simulink library "sm_wheel_loader_lib"  (R2025a)
settings: Solver=VariableStepAuto  StartTime=0.0  StopTime=10.0  RelTol=1e-3
undefined symbols (not defined in the file): AToTOrificeVector, BiPOrificeVector, boomHEArea, boomREArea, BToTOrificeVector, fluids, GRake, GToothL, GToothR, HMPST, HydFcnParams, logLoad, Position, PToAOrificeVector, PToBOrificeVector, RakeL, RakeR, testInput, Wheel_Loader, X, Y, Z
libraries: sm_lib x694, fl_lib x183, nesl_utility x74, SimscapeFluids_lib x62, sdl_lib x25, cvt_components_lib x25, simulink_extras x5, $bdroot x4, wheel_loader_contact_lib x4, ee_lib x2, SignalEditorBlockLib x1, batteryecm_lib x1
(part 12 of 26)

== system sm_wheel_loader_lib/Wheel Loader Vehicle/Frame Front/Lights/Cap Front ==
  Cap_Front : sm_lib/Body Elements/File Solid  ExtGeomFileName=FrameF_Cap_Front.step  UnitType=FromFile  ExtGeomFileUnits=m  StepReaderType=HEX  ExportConvexHullGeometry=off  InertiaType=Custom  BasedOnType=DensityFromFile  Density=1000  DensityUnits=kg/m^3  Mass=0.394195570353179  MassUnits=lbm  CenterOfMass=[0 18.9709186614173 25.112965984252]  CenterOfMassUnits=in  MomentsOfInertia=[0.29984658255218 0.29984658255218 0.584592682486173]  MomentsOfInertiaUnits=lbm*in^2  ProductsOfInertia=[0 0 0]  ProductsOfInertiaUnits=lbm*in^2  GraphicType=FromGeometry  MarkerShape=Sphere  MarkerSize=10  GraphicVisPropType=SimpleVisualProperties  GraphicDiffuseColor=[0.196078431 0.196078431 0.196078431]  GraphicOpacity=HMPST.Vis.Cap.opc  GraphicSpecularColor=[0.5 0.5 0.5 1.0]  GraphicAmbientColor=[0.15 0.15 0.15 1.0]  GraphicEmissiveColor=[0.0 0.0 0.0 1.0]  GraphicShininess=75  DoExposeReferenceFrame=on  SerializedFrames=<Frames/>
  Transform : sm_lib/Frames and Transforms/Rigid Transform  RotationMethod=ArbitraryAxis  FollAlignAxisA=+X  BaseAlignAxisA=+Y  FollAlignAxisB=+Y  BaseAlignAxisB=+Z  RotationStandardAxis=+Z  RotationAngle=0  RotationAngleUnits=rad  RotationArbitraryAxis=[0 0 0]  RotationSequenceAxes=FollowerAxes  RotationSequence=XYX  RotationSequenceAngles=[0 0 0]  RotationSequenceAnglesUnits=deg  RotationMatrix=[1 0 0; 0 1 0; 0 0 1]  Quaternion=[1 0 0 0]  TranslationMethod=Cartesian  TranslationCartesianOffset=[0 18.9709186614173 25.1378139370079]  TranslationCartesianOffsetUnits=in  TranslationStandardAxis=+Z  TranslationStandardOffset=0  TranslationStandardOffsetUnits=m  TranslationROffset=0  TranslationROffsetUnits=m  TranslationThetaOffset=0  TranslationThetaOffsetUnits=deg  TranslationZOffset=0  TranslationZOffsetUnits=m
  F : PMIOPort  Side=Left
  connections:
  Transform/RConn1 -- F/RConn1
  Cap_Front/RConn1 -- Transform/LConn1

== system sm_wheel_loader_lib/Wheel Loader Vehicle/Frame Front/Lights/Cap Side ==
  Cap_Side : sm_lib/Body Elements/File Solid  ExtGeomFileName=FrameF_Cap_Side.step  UnitType=FromFile  ExtGeomFileUnits=m  StepReaderType=HEX  ExportConvexHullGeometry=off  InertiaType=Custom  BasedOnType=DensityFromFile  Density=1000  DensityUnits=kg/m^3  Mass=0.326703632602991  MassUnits=lbm  CenterOfMass=[13.2699581496063 13.7324941732283 22.6905788976378]  CenterOfMassUnits=in  MomentsOfInertia=[0.25784270557939 0.189027697893249 0.286762231353936]  MomentsOfInertiaUnits=lbm*in^2  ProductsOfInertia=[0 0.0820087083851274 0]  ProductsOfInertiaUnits=lbm*in^2  GraphicType=FromGeometry  MarkerShape=Sphere  MarkerSize=10  GraphicVisPropType=SimpleVisualProperties  GraphicDiffuseColor=[0.901960784 0.901960784 0.901960784]  GraphicOpacity=HMPST.Vis.Cap.opc  GraphicSpecularColor=[0.5 0.5 0.5 1.0]  GraphicAmbientColor=[0.15 0.15 0.15 1.0]  GraphicEmissiveColor=[0.0 0.0 0.0 1.0]  GraphicShininess=75  DoExposeReferenceFrame=on  SerializedFrames=<Frames/>
  Transform : sm_lib/Frames and Transforms/Rigid Transform  RotationMethod=ArbitraryAxis  FollAlignAxisA=+X  BaseAlignAxisA=+Y  FollAlignAxisB=+Y  BaseAlignAxisB=+Z  RotationStandardAxis=+Z  RotationAngle=0  RotationAngleUnits=rad  RotationArbitraryAxis=[0 0 0]  RotationSequenceAxes=FollowerAxes  RotationSequence=XYX  RotationSequenceAngles=[0 0 0]  RotationSequenceAnglesUnits=deg  RotationMatrix=[1 0 0; 0 1 0; 0 0 1]  Quaternion=[1 0 0 0]  TranslationMethod=Cartesian  TranslationCartesianOffset=[29.4805690551181 -102.631127086614 57.6446281496063]  TranslationCartesianOffsetUnits=in  TranslationStandardAxis=+Z  TranslationStandardOffset=0  TranslationStandardOffsetUnits=m  TranslationROffset=0  TranslationROffsetUnits=m  TranslationThetaOffset=0  TranslationThetaOffsetUnits=deg  TranslationZOffset=0  TranslationZOffsetUnits=m
  G : PMIOPort  Side=Left
  connections:
  Transform/LConn1 -- G/RConn1
  Cap_Side/RConn1 -- Transform/RConn1

== system sm_wheel_loader_lib/Wheel Loader Vehicle/Frame Front/Lights/Light Left ==
  Housing : sm_lib/Body Elements/File Solid  ExtGeomFileName=LightF_Housing.step  UnitType=FromFile  ExtGeomFileUnits=m  StepReaderType=HEX  ExportConvexHullGeometry=off  InertiaType=Custom  BasedOnType=DensityFromFile  Density=1000  DensityUnits=kg/m^3  Mass=5.82907417512336  MassUnits=lbm  CenterOfMass=[-16.4284857874016 16.6341196850394 33.5621000393701]  CenterOfMassUnits=in  MomentsOfInertia=[45.900348235786 54.0150653364011 28.9269786264561]  MomentsOfInertiaUnits=lbm*in^2  ProductsOfInertia=[2.18871568666261 0.00164024251114051 -0.000652679832557995]  ProductsOfInertiaUnits=lbm*in^2  GraphicType=FromGeometry  MarkerShape=Sphere  MarkerSize=10  GraphicVisPropType=SimpleVisualProperties  GraphicDiffuseColor=[0.196078431 0.196078431 0.196078431]  GraphicOpacity=HMPST.Vis.Light.opc  GraphicSpecularColor=[0.5 0.5 0.5 1.0]  GraphicAmbientColor=[0.15 0.15 0.15 1.0]  GraphicEmissiveColor=[0.0 0.0 0.0 1.0]  GraphicShininess=75  DoExposeReferenceFrame=on  SerializedFrames=<Frames/>
  Inner_Reflector : sm_lib/Body Elements/File Solid  ExtGeomFileName=LightF_Inner_Reflector.step  UnitType=FromFile  ExtGeomFileUnits=m  StepReaderType=HEX  ExportConvexHullGeometry=off  InertiaType=Custom  BasedOnType=DensityFromFile  Density=1000  DensityUnits=kg/m^3  Mass=2.3813985010374  MassUnits=lbm  CenterOfMass=[-16.4286011417323 16.7992054724409 33.5198841732283]  CenterOfMassUnits=in  MomentsOfInertia=[16.7215889666979 21.0139771829924 9.91006504421532]  MomentsOfInertiaUnits=lbm*in^2  ProductsOfInertia=[0.553287970726677 -0.00263122236162124 0.000146938391623004]  ProductsOfInertiaUnits=lbm*in^2  GraphicType=FromGeometry  MarkerShape=Sphere  MarkerSize=10  GraphicVisPropType=SimpleVisualProperties  GraphicDiffuseColor=[1 1 1]  GraphicOpacity=HMPST.Vis.Light.opc  GraphicSpecularColor=[0.5 0.5 0.5 1.0]  GraphicAmbientColor=[0.15 0.15 0.15 1.0]  GraphicEmissiveColor=[0.0 0.0 0.0 1.0]  GraphicShininess=75  DoExposeReferenceFrame=on  SerializedFrames=<Frames/>
  Lens_Lower : sm_lib/Body Elements/File Solid  ExtGeomFileName=LightF_Lens_Lower.step  UnitType=FromFile  ExtGeomFileUnits=m  StepReaderType=HEX  ExportConvexHullGeometry=off  InertiaType=Custom  BasedOnType=DensityFromFile  Density=1000  DensityUnits=kg/m^3  Mass=0.955755653473624  MassUnits=lbm  CenterOfMass=[-16.4285714566929 18.8369745669291 32.0841470472441]  CenterOfMassUnits=in  MomentsOfInertia=[4.86310718087393 7.40813821570663 2.55427790198926]  MomentsOfInertiaUnits=lbm*in^2  ProductsOfInertia=[0.0290562126504745 0.000252870720467496 1.36686875928376e-05]  ProductsOfInertiaUnits=lbm*in^2  GraphicType=FromGeometry  MarkerShape=Sphere  MarkerSize=10  GraphicVisPropType=SimpleVisualProperties  GraphicDiffuseColor=[0.701960784 0.701960784 0.701960784]  GraphicOpacity=HMPST.Vis.Light.opc  GraphicSpecularColor=[0.5 0.5 0.5 1.0]  GraphicAmbientColor=[0.15 0.15 0.15 1.0]  GraphicEmissiveColor=[0.0 0.0 0.0 1.0]  GraphicShininess=75  DoExposeReferenceFrame=on  SerializedFrames=<Frames/>
  Lens_Upper : sm_lib/Body Elements/File Solid  ExtGeomFileName=LightF_Lens_Upper.step  UnitType=FromFile  ExtGeomFileUnits=m  StepReaderType=HEX  ExportConvexHullGeometry=off  InertiaType=Custom  BasedOnType=DensityFromFile  Density=1000  DensityUnits=kg/m^3  Mass=0.688422318479475  MassUnits=lbm  CenterOfMass=[-16.4285475590551 18.8615080708661 35.1565936614173]  CenterOfMassUnits=in  MomentsOfInertia=[0.831387671318652 2.25205980213972 1.42246614606763]  MomentsOfInertiaUnits=lbm*in^2  ProductsOfInertia=[0 -6.8343437964188e-06 0]  ProductsOfInertiaUnits=lbm*in^2  GraphicType=FromGeometry  MarkerShape=Sphere  MarkerSize=10  GraphicVisPropType=SimpleVisualProperties  GraphicDiffuseColor=[0.901960784 0.901960784 0.901960784]  GraphicOpacity=HMPST.Vis.Lens.opc  GraphicSpecularColor=[0.5 0.5 0.5 1.0]  GraphicAmbientColor=[0.15 0.15 0.15 1.0]  GraphicEmissiveColor=[0.0 0.0 0.0 1.0]  GraphicShininess=75  DoExposeReferenceFrame=on  SerializedFrames=<Frames/>
  Transform{,1..3} (4 alike) : sm_lib/Frames and Transforms/Rigid Transform  RotationMethod=ArbitraryAxis  FollAlignAxisA=+X  BaseAlignAxisA=+Y  FollAlignAxisB=+Y  BaseAlignAxisB=+Z  RotationStandardAxis=+Z  RotationAngle=0  RotationAngleUnits=rad  RotationArbitraryAxis=[0 0 0]  RotationSequenceAxes=FollowerAxes  RotationSequence=XYX  RotationSequenceAngles=[0 0 0]  RotationSequenceAnglesUnits=deg  RotationMatrix=[1 0 0; 0 1 0; 0 0 1]  Quaternion=[1 0 0 0]  TranslationMethod=Cartesian  TranslationCartesianOffset=[29.4805690551181 -102.631127086614 57.6446281496063]  TranslationCartesianOffsetUnits=in  TranslationStandardAxis=+Z  TranslationStandardOffset=0  TranslationStandardOffsetUnits=m  TranslationROffset=0  TranslationROffsetUnits=m  TranslationThetaOffset=0  TranslationThetaOffsetUnits=deg  TranslationZOffset=0  TranslationZOffsetUnits=m
  Transform4 : sm_lib/Frames and Transforms/Rigid Transform  RotationMethod=ArbitraryAxis  FollAlignAxisA=+X  BaseAlignAxisA=+Y  FollAlignAxisB=+Y  BaseAlignAxisB=+Z  RotationStandardAxis=+Z  RotationAngle=1.5707963267949  RotationAngleUnits=rad  RotationArbitraryAxis=[-1 0 0]  RotationSequenceAxes=FollowerAxes  RotationSequence=XYX  RotationSequenceAngles=[0 0 0]  RotationSequenceAnglesUnits=deg  RotationMatrix=[1 0 0; 0 1 0; 0 0 1]  Quaternion=[1 0 0 0]  TranslationMethod=Cartesian  TranslationCartesianOffset=[-16.4285533858268 13.4490081889764 34.3374097244095]  TranslationCartesianOffsetUnits=in  TranslationStandardAxis=+Z  TranslationStandardOffset=0  TranslationStandardOffsetUnits=m  TranslationROffset=0  TranslationROffsetUnits=m  TranslationThetaOffset=0  TranslationThetaOffsetUnits=deg  TranslationZOffset=0  TranslationZOffsetUnits=m
  F : PMIOPort  Side=Left
  connections:
  Transform3/RConn1 -- Transform4/LConn1 -- Housing/RConn1
  Lens_Lower/RConn1 -- Transform2/RConn1
  Lens_Upper/RConn1 -- Transform1/RConn1
  Inner_Reflector/RConn1 -- Transform/RConn1
  Transform4/RConn1 -- F/RConn1
  Transform3/LConn1 -- Transform2/LConn1 -- Transform1/LConn1 -- Transform/LConn1

== system sm_wheel_loader_lib/Wheel Loader Vehicle/Frame Front/Lights/Light Right ==
  Inner_Reflector : sm_lib/Body Elements/File Solid  ExtGeomFileName=LightF_Inner_Reflector.step  UnitType=FromFile  ExtGeomFileUnits=m  StepReaderType=HEX  ExportConvexHullGeometry=off  InertiaType=Custom  BasedOnType=DensityFromFile  Density=1000  DensityUnits=kg/m^3  Mass=2.3813985010374  MassUnits=lbm  CenterOfMass=[-16.4286011417323 16.7992054724409 33.5198841732283]  CenterOfMassUnits=in  MomentsOfInertia=[16.7215889666979 21.0139771829924 9.91006504421532]  MomentsOfInertiaUnits=lbm*in^2  ProductsOfInertia=[0.553287970726677 -0.00263122236162124 0.000146938391623004]  ProductsOfInertiaUnits=lbm*in^2  GraphicType=FromGeometry  MarkerShape=Sphere  MarkerSize=10  GraphicVisPropType=SimpleVisualProperties  GraphicDiffuseColor=[1 1 1]  GraphicOpacity=HMPST.Vis.Light.opc  GraphicSpecularColor=[0.5 0.5 0.5 1.0]  GraphicAmbientColor=[0.15 0.15 0.15 1.0]  GraphicEmissiveColor=[0.0 0.0 0.0 1.0]  GraphicShininess=75  DoExposeReferenceFrame=on  SerializedFrames=<Frames/>
  Lens_Lower : sm_lib/Body Elements/File Solid  ExtGeomFileName=LightF_Lens_Lower.step  UnitType=FromFile  ExtGeomFileUnits=m  StepReaderType=HEX  ExportConvexHullGeometry=off  InertiaType=Custom  BasedOnType=DensityFromFile  Density=1000  DensityUnits=kg/m^3  Mass=0.955755653473624  MassUnits=lbm  CenterOfMass=[-16.4285714566929 18.8369745669291 32.0841470472441]  CenterOfMassUnits=in  MomentsOfInertia=[4.86310718087393 7.40813821570663 2.55427790198926]  MomentsOfInertiaUnits=lbm*in^2  ProductsOfInertia=[0.0290562126504745 0.000252870720467496 1.36686875928376e-05]  ProductsOfInertiaUnits=lbm*in^2  GraphicType=FromGeometry  MarkerShape=Sphere  MarkerSize=10  GraphicVisPropType=SimpleVisualProperties  GraphicDiffuseColor=[0.701960784 0.701960784 0.701960784]  GraphicOpacity=HMPST.Vis.Light.opc  GraphicSpecularColor=[0.5 0.5 0.5 1.0]  GraphicAmbientColor=[0.15 0.15 0.15 1.0]  GraphicEmissiveColor=[0.0 0.0 0.0 1.0]  GraphicShininess=75  DoExposeReferenceFrame=on  SerializedFrames=<Frames/>
  Lens_Upper : sm_lib/Body Elements/File Solid  ExtGeomFileName=LightF_Lens_Upper.step  UnitType=FromFile  ExtGeomFileUnits=m  StepReaderType=HEX  ExportConvexHullGeometry=off  InertiaType=Custom  BasedOnType=DensityFromFile  Density=1000  DensityUnits=kg/m^3  Mass=0.688422318479475  MassUnits=lbm  CenterOfMass=[-16.4285475590551 18.8615080708661 35.1565936614173]  CenterOfMassUnits=in  MomentsOfInertia=[0.831387671318652 2.25205980213972 1.42246614606763]  MomentsOfInertiaUnits=lbm*in^2  ProductsOfInertia=[0 -6.8343437964188e-06 0]  ProductsOfInertiaUnits=lbm*in^2  GraphicType=FromGeometry  MarkerShape=Sphere  MarkerSize=10  GraphicVisPropType=SimpleVisualProperties  GraphicDiffuseColor=[0.901960784 0.901960784 0.901960784]  GraphicOpacity=HMPST.Vis.Lens.opc  GraphicSpecularColor=[0.5 0.5 0.5 1.0]  GraphicAmbientColor=[0.15 0.15 0.15 1.0]  GraphicEmissiveColor=[0.0 0.0 0.0 1.0]  GraphicShininess=75  DoExposeReferenceFrame=on  SerializedFrames=<Frames/>
  Solid : sm_lib/Body Elements/File Solid  ExtGeomFileName=LightF_Housing.step  UnitType=FromFile  ExtGeomFileUnits=m  StepReaderType=HEX  ExportConvexHullGeometry=off  InertiaType=Custom  BasedOnType=DensityFromFile  Density=1000  DensityUnits=kg/m^3  Mass=5.82907417512336  MassUnits=lbm  CenterOfMass=[-16.4284857874016 16.6341196850394 33.5621000393701]  CenterOfMassUnits=in  MomentsOfInertia=[45.900348235786 54.0150653364011 28.9269786264561]  MomentsOfInertiaUnits=lbm*in^2  ProductsOfInertia=[2.18871568666261 0.00164024251114051 -0.000652679832557995]  ProductsOfInertiaUnits=lbm*in^2  GraphicType=FromGeometry  MarkerShape=Sphere  MarkerSize=10  GraphicVisPropType=SimpleVisualProperties  GraphicDiffuseColor=[0.196078431 0.196078431 0.196078431]  GraphicOpacity=HMPST.Vis.Light.opc  GraphicSpecularColor=[0.5 0.5 0.5 1.0]  GraphicAmbientColor=[0.15 0.15 0.15 1.0]  GraphicEmissiveColor=[0.0 0.0 0.0 1.0]  GraphicShininess=75  DoExposeReferenceFrame=on  SerializedFrames=<Frames/>
  Transform{,1..3} (4 alike) : sm_lib/Frames and Transforms/Rigid Transform  RotationMethod=ArbitraryAxis  FollAlignAxisA=+X  BaseAlignAxisA=+Y  FollAlignAxisB=+Y  BaseAlignAxisB=+Z  RotationStandardAxis=+Z  RotationAngle=0  RotationAngleUnits=rad  RotationArbitraryAxis=[0 0 0]  RotationSequenceAxes=FollowerAxes  RotationSequence=XYX  RotationSequenceAngles=[0 0 0]  RotationSequenceAnglesUnits=deg  RotationMatrix=[1 0 0; 0 1 0; 0 0 1]  Quaternion=[1 0 0 0]  TranslationMethod=Cartesian  TranslationCartesianOffset=[62.3376758661417 -102.631127086614 57.6446281496063]  TranslationCartesianOffsetUnits=in  TranslationStandardAxis=+Z  TranslationStandardOffset=0  TranslationStandardOffsetUnits=m  TranslationROffset=0  TranslationROffsetUnits=m  TranslationThetaOffset=0  TranslationThetaOffsetUnits=deg  TranslationZOffset=0  TranslationZOffsetUnits=m
  Transform4 : sm_lib/Frames and Transforms/Rigid Transform  RotationMethod=ArbitraryAxis  FollAlignAxisA=+X  BaseAlignAxisA=+Y  FollAlignAxisB=+Y  BaseAlignAxisB=+Z  RotationStandardAxis=+Z  RotationAngle=1.5707963267949  RotationAngleUnits=rad  RotationArbitraryAxis=[-1 0 0]  RotationSequenceAxes=FollowerAxes  RotationSequence=XYX  RotationSequenceAngles=[0 0 0]  RotationSequenceAnglesUnits=deg  RotationMatrix=[1 0 0; 0 1 0; 0 0 1]  Quaternion=[1 0 0 0]  TranslationMethod=Cartesian  TranslationCartesianOffset=[-16.4285533858268 13.4490081889764 34.3374097244095]  TranslationCartesianOffsetUnits=in  TranslationStandardAxis=+Z  TranslationStandardOffset=0  TranslationStandardOffsetUnits=m  TranslationROffset=0  TranslationROffsetUnits=m  TranslationThetaOffset=0  TranslationThetaOffsetUnits=deg  TranslationZOffset=0  TranslationZOffsetUnits=m
  F : PMIOPort  Side=Left
  connections:
  Transform4/LConn1 -- Transform3/RConn1 -- Solid/RConn1
  Inner_Reflector/RConn1 -- Transform2/RConn1
  Lens_Upper/RConn1 -- Transform1/RConn1
  Lens_Lower/RConn1 -- Transform/RConn1
  Transform4/RConn1 -- F/RConn1
  Transform3/LConn1 -- Transform2/LConn1 -- Transform1/LConn1 -- Transform/LConn1

== system sm_wheel_loader_lib/Wheel Loader Vehicle/Frame Rear/Handles Panels/Side Handles ==
  HandleL : sm_lib/Body Elements/File Solid  ExtGeomFileName=Cab_HandleL.step  UnitType=FromFile  ExtGeomFileUnits=m  StepReaderType=HEX  ExportConvexHullGeometry=off  InertiaType=Custom  BasedOnType=DensityFromFile  Density=1000  DensityUnits=kg/m^3  Mass=6.28305972166154  MassUnits=lbm  CenterOfMass=[-17.3045312204724 -39.1271442913386 31.4849240944882]  CenterOfMassUnits=in  MomentsOfInertia=[212.912574457631 25.500464180277 191.478835295835]  MomentsOfInertiaUnits=lbm*in^2  ProductsOfInertia=[38.7009923887161 4.44232346767222e-05 -0.000140104047826585]  ProductsOfInertiaUnits=lbm*in^2  GraphicType=FromGeometry  MarkerShape=Sphere  MarkerSize=10  GraphicVisPropType=SimpleVisualProperties  GraphicDiffuseColor=[0.301960784 0.301960784 0.301960784]  GraphicOpacity=HMPST.Vis.SeatTrim.opc  GraphicSpecularColor=[0.5 0.5 0.5 1.0]  GraphicAmbientColor=[0.15 0.15 0.15 1.0]  GraphicEmissiveColor=[0.0 0.0 0.0 1.0]  GraphicShininess=75  DoExposeReferenceFrame=on  SerializedFrames=<Frames/>
  HandleR : sm_lib/Body Elements/File Solid  ExtGeomFileName=Cab_HandleR.step  UnitType=FromFile  ExtGeomFileUnits=m  StepReaderType=HEX  ExportConvexHullGeometry=off  InertiaType=Custom  BasedOnType=DensityFromFile  Density=1000  DensityUnits=kg/m^3  Mass=6.28305972166154  MassUnits=lbm  CenterOfMass=[17.3045238976378 -39.1271442913386 31.4849240944882]  CenterOfMassUnits=in  MomentsOfInertia=[212.912574457631 25.500464180277 191.478835295835]  MomentsOfInertiaUnits=lbm*in^2  ProductsOfInertia=[38.7009923887161 4.44232346767222e-05 -0.000140104047826585]  ProductsOfInertiaUnits=lbm*in^2  GraphicType=FromGeometry  MarkerShape=Sphere  MarkerSize=10  GraphicVisPropType=SimpleVisualProperties  GraphicDiffuseColor=[0.301960784 0.301960784 0.301960784]  GraphicOpacity=HMPST.Vis.SeatTrim.opc  GraphicSpecularColor=[0.5 0.5 0.5 1.0]  GraphicAmbientColor=[0.15 0.15 0.15 1.0]  GraphicEmissiveColor=[0.0 0.0 0.0 1.0]  GraphicShininess=75  DoExposeReferenceFrame=on  SerializedFrames=<Frames/>
  Transform : sm_lib/Frames and Transforms/Rigid Transform  RotationMethod=ArbitraryAxis  FollAlignAxisA=+X  BaseAlignAxisA=+Y  FollAlignAxisB=+Y  BaseAlignAxisB=+Z  RotationStandardAxis=+Z  RotationAngle=0  RotationAngleUnits=rad  RotationArbitraryAxis=[0 0 0]  RotationSequenceAxes=FollowerAxes  RotationSequence=XYX  RotationSequenceAngles=[0 0 0]  RotationSequenceAnglesUnits=deg  RotationMatrix=[1 0 0; 0 1 0; 0 0 1]  Quaternion=[1 0 0 0]  TranslationMethod=Cartesian  TranslationCartesianOffset=[-7.89410114173228 5.59542992125984 -19.0696908267717]  TranslationCartesianOffsetUnits=in  TranslationStandardAxis=+Z  TranslationStandardOffset=0  TranslationStandardOffsetUnits=m  TranslationROffset=0  TranslationROffsetUnits=m  TranslationThetaOffset=0  TranslationThetaOffsetUnits=deg  TranslationZOffset=0  TranslationZOffsetUnits=m
  Transform1 : sm_lib/Frames and Transforms/Rigid Transform  RotationMethod=ArbitraryAxis  FollAlignAxisA=+X  BaseAlignAxisA=+Y  FollAlignAxisB=+Y  BaseAlignAxisB=+Z  RotationStandardAxis=+Z  RotationAngle=0.218166156574323  RotationAngleUnits=rad  RotationArbitraryAxis=[-1 0 0]  RotationSequenceAxes=FollowerAxes  RotationSequence=XYX  RotationSequenceAngles=[0 0 0]  RotationSequenceAnglesUnits=deg  RotationMatrix=[1 0 0; 0 1 0; 0 0 1]  Quaternion=[1 0 0 0]  TranslationMethod=Cartesian  TranslationCartesianOffset=[-17.3045275590551 -39.3975186614173 30.2634644094488]  TranslationCartesianOffsetUnits=in  TranslationStandardAxis=+Z  TranslationStandardOffset=0  TranslationStandardOffsetUnits=m  TranslationROffset=0  TranslationROffsetUnits=m  TranslationThetaOffset=0  TranslationThetaOffsetUnits=deg  TranslationZOffset=0  TranslationZOffsetUnits=m
  Transform2 : sm_lib/Frames and Transforms/Rigid Transform  RotationMethod=ArbitraryAxis  FollAlignAxisA=+X  BaseAlignAxisA=+Y  FollAlignAxisB=+Y  BaseAlignAxisB=+Z  RotationStandardAxis=+Z  RotationAngle=0  RotationAngleUnits=rad  RotationArbitraryAxis=[0 0 0]  RotationSequenceAxes=FollowerAxes  RotationSequence=XYX  RotationSequenceAngles=[0 0 0]  RotationSequenceAnglesUnits=deg  RotationMatrix=[1 0 0; 0 1 0; 0 0 1]  Quaternion=[1 0 0 0]  TranslationMethod=Cartesian  TranslationCartesianOffset=[-7.89410114173228 5.59542992125984 -19.0696908267717]  TranslationCartesianOffsetUnits=in  TranslationStandardAxis=+Z  TranslationStandardOffset=0  TranslationStandardOffsetUnits=m  TranslationROffset=0  TranslationROffsetUnits=m  TranslationThetaOffset=0  TranslationThetaOffsetUnits=deg  TranslationZOffset=0  TranslationZOffsetUnits=m
  F : PMIOPort  Side=Left
  connections:
  Transform2/RConn1 -- HandleL/RConn1 -- Transform1/LConn1
  HandleR/RConn1 -- Transform/RConn1
  Transform1/RConn1 -- F/RConn1
  Transform2/LConn1 -- Transform/LConn1

== system sm_wheel_loader_lib/Wheel Loader Vehicle/Frame Rear/Handles Panels/Side Panels ==
  SeatTrimOuterL : sm_lib/Body Elements/File Solid  ExtGeomFileName=Cab_SeatTrimOuterL.step  UnitType=FromFile  ExtGeomFileUnits=m  StepReaderType=HEX  ExportConvexHullGeometry=off  InertiaType=Custom  BasedOnType=DensityFromFile  Density=1000  DensityUnits=kg/m^3  Mass=4.87052143315374  MassUnits=lbm  CenterOfMass=[-19.8295275590551 -43.9655751574803 25.4392532283465]  CenterOfMassUnits=in  MomentsOfInertia=[209.666978760431 31.2673620706489 178.412297814697]  MomentsOfInertiaUnits=lbm*in^2  ProductsOfInertia=[-6.07990400190403 0 0]  ProductsOfInertiaUnits=lbm*in^2  GraphicType=FromGeometry  MarkerShape=Sphere  MarkerSize=10  GraphicVisPropType=SimpleVisualProperties  GraphicDiffuseColor=[0.196078431 0.196078431 0.196078431]  GraphicOpacity=HMPST.Vis.SeatTrim.opc  GraphicSpecularColor=[0.5 0.5 0.5 1.0]  GraphicAmbientColor=[0.15 0.15 0.15 1.0]  GraphicEmissiveColor=[0.0 0.0 0.0 1.0]  GraphicShininess=75  DoExposeReferenceFrame=on  SerializedFrames=<Frames/>
  SeatTrimOuterR : sm_lib/Body Elements/File Solid  ExtGeomFileName=Cab_SeatTrimOuterR.step  UnitType=FromFile  ExtGeomFileUnits=m  StepReaderType=HEX  ExportConvexHullGeometry=off  InertiaType=Custom  BasedOnType=DensityFromFile  Density=1000  DensityUnits=kg/m^3  Mass=4.87052143315374  MassUnits=lbm  CenterOfMass=[19.8295275590551 -43.9655751574803 25.4392532283465]  CenterOfMassUnits=in  MomentsOfInertia=[209.666978760431 31.2673620706489 178.412297814697]  MomentsOfInertiaUnits=lbm*in^2  ProductsOfInertia=[-6.07990400190403 0 0]  ProductsOfInertiaUnits=lbm*in^2  GraphicType=FromGeometry  MarkerShape=Sphere  MarkerSize=10  GraphicVisPropType=SimpleVisualProperties  GraphicDiffuseColor=[0.196078431 0.196078431 0.196078431]  GraphicOpacity=HMPST.Vis.SeatTrim.opc  GraphicSpecularColor=[0.5 0.5 0.5 1.0]  GraphicAmbientColor=[0.15 0.15 0.15 1.0]  GraphicEmissiveColor=[0.0 0.0 0.0 1.0]  GraphicShininess=75  DoExposeReferenceFrame=on  SerializedFrames=<Frames/>
  Transform : sm_lib/Frames and Transforms/Rigid Transform  RotationMethod=ArbitraryAxis  FollAlignAxisA=+X  BaseAlignAxisA=+Y  FollAlignAxisB=+Y  BaseAlignAxisB=+Z  RotationStandardAxis=+Z  RotationAngle=0  RotationAngleUnits=rad  RotationArbitraryAxis=[0 0 0]  RotationSequenceAxes=FollowerAxes  RotationSequence=XYX  RotationSequenceAngles=[0 0 0]  RotationSequenceAnglesUnits=deg  RotationMatrix=[1 0 0; 0 1 0; 0 0 1]  Quaternion=[1 0 0 0]  TranslationMethod=Cartesian  TranslationCartesianOffset=[-7.89410114173228 5.59542992125984 -19.0696908267717]  TranslationCartesianOffsetUnits=in  TranslationStandardAxis=+Z  TranslationStandardOffset=0  TranslationStandardOffsetUnits=m  TranslationROffset=0  TranslationROffsetUnits=m  TranslationThetaOffset=0  TranslationThetaOffsetUnits=deg  TranslationZOffset=0  TranslationZOffsetUnits=m
  Transform1 : sm_lib/Frames and Transforms/Rigid Transform  RotationMethod=ArbitraryAxis  FollAlignAxisA=+X  BaseAlignAxisA=+Y  FollAlignAxisB=+Y  BaseAlignAxisB=+Z  RotationStandardAxis=+Z  RotationAngle=2.0943951023932  RotationAngleUnits=rad  RotationArbitraryAxis=[0.577350269189626 0.577350269189626 0.577350269189626]  RotationSequenceAxes=FollowerAxes  RotationSequence=XYX  RotationSequenceAngles=[0 0 0]  RotationSequenceAnglesUnits=deg  RotationMatrix=[1 0 0; 0 1 0; 0 0 1]  Quaternion=[1 0 0 0]  TranslationMethod=Cartesian  TranslationCartesianOffset=[19.7670275590551 -43.9655751574803 25.4392532283465]  TranslationCartesianOffsetUnits=in  TranslationStandardAxis=+Z  TranslationStandardOffset=0  TranslationStandardOffsetUnits=m  TranslationROffset=0  TranslationROffsetUnits=m  TranslationThetaOffset=0  TranslationThetaOffsetUnits=deg  TranslationZOffset=0  TranslationZOffsetUnits=m
  Transform2 : sm_lib/Frames and Transforms/Rigid Transform  RotationMethod=ArbitraryAxis  FollAlignAxisA=+X  BaseAlignAxisA=+Y  FollAlignAxisB=+Y  BaseAlignAxisB=+Z  RotationStandardAxis=+Z  RotationAngle=0  RotationAngleUnits=rad  RotationArbitraryAxis=[0 0 0]  RotationSequenceAxes=FollowerAxes  RotationSequence=XYX  RotationSequenceAngles=[0 0 0]  RotationSequenceAnglesUnits=deg  RotationMatrix=[1 0 0; 0 1 0; 0 0 1]  Quaternion=[1 0 0 0]  TranslationMethod=Cartesian  TranslationCartesianOffset=[-7.89410114173228 5.59542992125984 -19.0696908267717]  TranslationCartesianOffsetUnits=in  TranslationStandardAxis=+Z  TranslationStandardOffset=0  TranslationStandardOffsetUnits=m  TranslationROffset=0  TranslationROffsetUnits=m  TranslationThetaOffset=0  TranslationThetaOffsetUnits=deg  TranslationZOffset=0  TranslationZOffsetUnits=m
  F : PMIOPort  Side=Left
  connections:
  Transform2/RConn1 -- Transform1/LConn1 -- SeatTrimOuterR/RConn1
  SeatTrimOuterL/RConn1 -- Transform/RConn1
  Transform1/RConn1 -- F/RConn1
  Transform2/LConn1 -- Transform/LConn1

== system sm_wheel_loader_lib/Wheel Loader Vehicle/Linkage/Implement/Bucket ==
  Bus Element In1 : Inport  PortName=Cmd
  Bucket : Subsystem  Tag=97CFEBBA-90A8-4A4C-AFF6-5F2FCDFBD586
      mask Display: image('sm_wheel_loader_vehicle_bucket_IMAGE.png')
  Bus Creator : BusCreator  Inputs=7
  Constant{,1..6} (7 alike) : Constant  Value=0
  Simscape Bus : SimscapeBus  HierarchyStrings=Bottom
  Terminator : Terminator
  Act : PMIOPort  Side=Right
  Link : PMIOPort  Port=2  Side=Left
  Arm : PMIOPort  Port=3  Side=Left
  GImpl : PMIOPort  Port=4  Side=Right
  m : Outport
  wires:
  Constant5/1 -> Bus Creator/2  "vL"
  Constant6/1 -> Bus Creator/6  "vR"
  Constant4/1 -> Bus Creator/7  "pR"
  Bus Creator/1 -> m/1
  Constant3/1 -> Bus Creator/3  "pL"
  Constant2/1 -> Bus Creator/4  "power"
  Constant1/1 -> Bus Creator/5  "forceR"
  Constant/1 -> Bus Creator/1  "forceL"
  Bus Element In1/1 -> Terminator/1
  connections:
  Bucket/RConn1 -- Simscape Bus/LConn1
  GImpl/RConn1 -- Simscape Bus/RConn1
  Arm/RConn1 -- Bucket/LConn2
  Bucket/LConn1 -- Link/RConn1

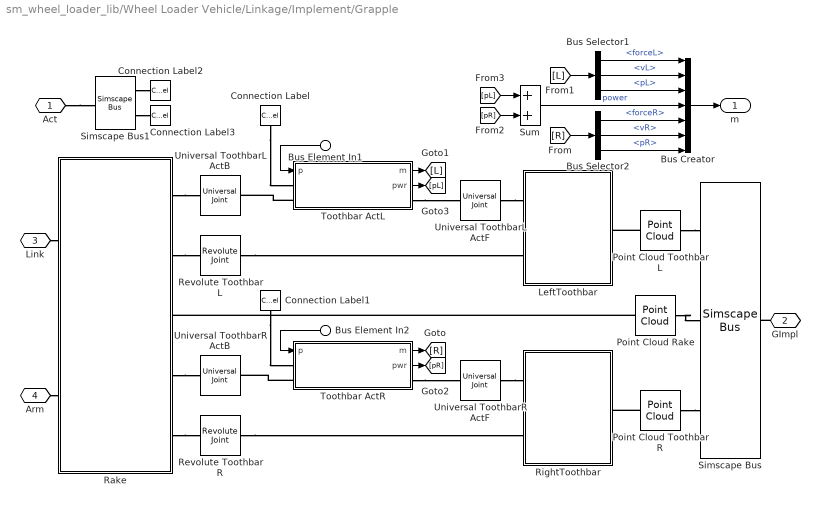
== system sm_wheel_loader_lib/Wheel Loader Vehicle/Linkage/Implement/Grapple ==
  Bus Element In1 : Inport  PortName=Cmd
  Bus Element In2 : Inport  PortName=Cmd
  Bus Creator : BusCreator  Inputs=7
  Bus Selector1 : BusSelector  OutputSignals=forceL,vL,pL
  Bus Selector2 : BusSelector  OutputSignals=forceR,vR,pR
  Connection Label : ConnectionLabel  Label=RL
  Connection Label1 : ConnectionLabel  Label=RR
  Connection Label2 : ConnectionLabel  Label=RL
  Connection Label3 : ConnectionLabel  Label=RR
  LeftToothbar : Subsystem  Tag=ACE2EE0B-C71A-8645-8B11-A2CDF5242645
      mask Display: image('sm_wheel_loader_vehicle_linkage_rakeTooth_IMAGE.png');
  Point Cloud Rake : sm_lib/Curves and Surfaces/Point Cloud  CoordinatesMatrix=HMPST.Grapple.ptcld.rake  CoordinatesMatrixUnits=m  GraphicType=MarkerCloud  GraphicSphereRadius=0.01  GraphicSphereRadiusUnits=m  GraphicVisPropType=SimpleVisualProperties  GraphicDiffuseColor=[0 0 1]  GraphicOpacity=1.0  GraphicSpecularColor=[0.5 0.5 0.5 1.0]  GraphicAmbientColor=[0.15 0.15 0.15 1.0]  GraphicEmissiveColor=[0.0 0.0 0.0 1.0]  GraphicShininess=75
  Point Cloud Toothbar L : sm_lib/Curves and Surfaces/Point Cloud  CoordinatesMatrix=HMPST.Grapple.ptcld.toothL  CoordinatesMatrixUnits=m  GraphicType=MarkerCloud  GraphicSphereRadius=0.01  GraphicSphereRadiusUnits=m  GraphicVisPropType=SimpleVisualProperties  GraphicDiffuseColor=[0 0 1]  GraphicOpacity=1.0  GraphicSpecularColor=[0.5 0.5 0.5 1.0]  GraphicAmbientColor=[0.15 0.15 0.15 1.0]  GraphicEmissiveColor=[0.0 0.0 0.0 1.0]  GraphicShininess=75
  Point Cloud Toothbar R : sm_lib/Curves and Surfaces/Point Cloud  CoordinatesMatrix=HMPST.Grapple.ptcld.toothR  CoordinatesMatrixUnits=m  GraphicType=MarkerCloud  GraphicSphereRadius=0.01  GraphicSphereRadiusUnits=m  GraphicVisPropType=SimpleVisualProperties  GraphicDiffuseColor=[0 0 1]  GraphicOpacity=1.0  GraphicSpecularColor=[0.5 0.5 0.5 1.0]  GraphicAmbientColor=[0.15 0.15 0.15 1.0]  GraphicEmissiveColor=[0.0 0.0 0.0 1.0]  GraphicShininess=75
  Rake : Subsystem
      mask Display: image('sm_wheel_loader_vehicle_linkage_Rake_IMAGE.png')
  Revolute Toothbar L : sm_lib/Joints/Revolute Joint  JointMode=Normal  CompositeWrenchDir=FollowerOnBase  CompositeWrenchFrame=BaseFrame  SenseConstraintForce=off  SenseConstraintTorque=off  SenseTotalForce=off  SenseTotalTorque=off  PositionTargetSpecify=off  PositionTargetPriority=High  PositionTargetValue=0  PositionTargetValueUnits=deg  VelocityTargetSpecify=off  VelocityTargetPriority=High  VelocityTargetValue=0  VelocityTargetValueUnits=deg/s  EquilibriumPosition=0  EquilibriumPositionUnits=deg  SpringStiffness=0  SpringStiffnessUnits=N*m/deg  DampingCoefficient=0  DampingCoefficientUnits=N*m/(deg/s)  LowerLimitSpecify=off  LowerLimitBound=-90  LowerLimitBoundUnits=deg  LowerLimitStiffness=1e4  LowerLimitStiffnessUnits=N*m/deg  LowerLimitDamping=10  LowerLimitDampingUnits=N*m/(deg/s)  LowerLimitTransitionRegionWidth=0.1  LowerLimitTransitionRegionWidthUnits=deg  UpperLimitSpecify=off  UpperLimitBound=90  UpperLimitBoundUnits=deg  UpperLimitStiffness=1e4  UpperLimitStiffnessUnits=N*m/deg  UpperLimitDamping=10  UpperLimitDampingUnits=N*m/(deg/s)  UpperLimitTransitionRegionWidth=0.1  UpperLimitTransitionRegionWidthUnits=deg  TorqueActuationMode=NoTorque  MotionActuationMode=ComputedMotion  SensePosition=off  SenseVelocity=off  SenseAcceleration=off  SenseTorqueForce=off  SenseLowerLimitTorqueForce=off  SenseUpperLimitTorqueForce=off
  Revolute Toothbar R : sm_lib/Joints/Revolute Joint  JointMode=Normal  CompositeWrenchDir=FollowerOnBase  CompositeWrenchFrame=BaseFrame  SenseConstraintForce=off  SenseConstraintTorque=off  SenseTotalForce=off  SenseTotalTorque=off  PositionTargetSpecify=off  PositionTargetPriority=High  PositionTargetValue=0  PositionTargetValueUnits=deg  VelocityTargetSpecify=off  VelocityTargetPriority=High  VelocityTargetValue=0  VelocityTargetValueUnits=deg/s  EquilibriumPosition=0  EquilibriumPositionUnits=deg  SpringStiffness=0  SpringStiffnessUnits=N*m/deg  DampingCoefficient=0  DampingCoefficientUnits=N*m/(deg/s)  LowerLimitSpecify=off  LowerLimitBound=-90  LowerLimitBoundUnits=deg  LowerLimitStiffness=1e4  LowerLimitStiffnessUnits=N*m/deg  LowerLimitDamping=10  LowerLimitDampingUnits=N*m/(deg/s)  LowerLimitTransitionRegionWidth=0.1  LowerLimitTransitionRegionWidthUnits=deg  UpperLimitSpecify=off  UpperLimitBound=90  UpperLimitBoundUnits=deg  UpperLimitStiffness=1e4  UpperLimitStiffnessUnits=N*m/deg  UpperLimitDamping=10  UpperLimitDampingUnits=N*m/(deg/s)  UpperLimitTransitionRegionWidth=0.1  UpperLimitTransitionRegionWidthUnits=deg  TorqueActuationMode=NoTorque  MotionActuationMode=ComputedMotion  SensePosition=off  SenseVelocity=off  SenseAcceleration=off  SenseTorqueForce=off  SenseLowerLimitTorqueForce=off  SenseUpperLimitTorqueForce=off
  RightToothbar : Subsystem  Tag=9CEF6292-F94B-A247-8261-D122692AABCF
      mask Display: image('sm_wheel_loader_vehicle_linkage_rakeTooth_IMAGE.png')
  Simscape Bus : SimscapeBus  HierarchyStrings=GToothL;GRake;GToothR
  Simscape Bus1 : SimscapeBus  HierarchyStrings=RakeL;RakeR
  Sum : Sum
  Toothbar ActL : Subsystem  Tag=f9ac6c41-a333-4287-85b5-ec7c60937c4d  mask{popup_actuator_model=Position}
      mask prompts: popup_actuator_model "Actuator Mode"
      mask init:
      | if(strcmp(get_param(gcb,'popup_actuator_model'),'Shaft'))
      |     set_param([gcb '/Actuator'],'LabelModeActiveChoice','Shaft')
      | else
      |     set_param([gcb '/Actuator'],'LabelModeActiveChoice','Position')
      | end
      mask TypeOptions popup_actuator_model: Shaft | Position
      mask Display:
      | if(strcmp(get_param(gcb,'popup_actuator_model'),'Position'))
      |     image('sm_wheel_loader_actuator_intfPosition_IMAGE.png')
      | else
      |     image('sm_wheel_loader_actuator_intfShaft_IMAGE.png')
      | end
  Toothbar ActR : Subsystem  Tag=351c651f-b42b-4eb7-b667-a38245ac79b1  mask{popup_actuator_model=Position}
      mask prompts: popup_actuator_model "Actuator Mode"
      mask init:
      | if(strcmp(get_param(gcb,'popup_actuator_model'),'Shaft'))
      |     set_param([gcb '/Actuator'],'LabelModeActiveChoice','Shaft')
      | else
      |     set_param([gcb '/Actuator'],'LabelModeActiveChoice','Position')
      | end
      mask TypeOptions popup_actuator_model: Shaft | Position
      mask Display:
      | if(strcmp(get_param(gcb,'popup_actuator_model'),'Position'))
      |     image('sm_wheel_loader_actuator_intfPosition_IMAGE.png')
      | else
      |     image('sm_wheel_loader_actuator_intfShaft_IMAGE.png')
      | end
  Universal ToothbarL ActB : sm_lib/Joints/Universal Joint  JointMode=Normal  CompositeWrenchDir=FollowerOnBase  CompositeWrenchFrame=BaseFrame  SenseConstraintForce=off  SenseConstraintTorque=off  SenseTotalForce=off  SenseTotalTorque=off  RxPositionTargetSpecify=off  RxPositionTargetPriority=High  RxPositionTargetValue=0  RxPositionTargetValueUnits=deg  RxVelocityTargetSpecify=off  RxVelocityTargetPriority=High  RxVelocityTargetValue=0  RxVelocityTargetValueUnits=deg/s  RxEquilibriumPosition=0  RxEquilibriumPositionUnits=deg  RxSpringStiffness=0  RxSpringStiffnessUnits=N*m/deg  RxDampingCoefficient=0  RxDampingCoefficientUnits=N*m/(deg/s)  RxLowerLimitSpecify=off  RxLowerLimitBound=-90  RxLowerLimitBoundUnits=deg  RxLowerLimitStiffness=1e4  RxLowerLimitStiffnessUnits=N*m/deg  RxLowerLimitDamping=10  RxLowerLimitDampingUnits=N*m/(deg/s)  RxLowerLimitTransitionRegionWidth=0.1  RxLowerLimitTransitionRegionWidthUnits=deg  RxUpperLimitSpecify=off  RxUpperLimitBound=90  RxUpperLimitBoundUnits=deg  RxUpperLimitStiffness=1e4  RxUpperLimitStiffnessUnits=N*m/deg  RxUpperLimitDamping=10  RxUpperLimitDampingUnits=N*m/(deg/s)  RxUpperLimitTransitionRegionWidth=0.1  RxUpperLimitTransitionRegionWidthUnits=deg  RxTorqueActuationMode=NoTorque  RxMotionActuationMode=ComputedMotion  RxSensePosition=off  RxSenseVelocity=off  RxSenseAcceleration=off  RxSenseTorqueForce=off  RxSenseLowerLimitTorqueForce=off  RxSenseUpperLimitTorqueForce=off  RyPositionTargetSpecify=off  RyPositionTargetPriority=High  RyPositionTargetValue=0  RyPositionTargetValueUnits=deg  RyVelocityTargetSpecify=off  RyVelocityTargetPriority=High  RyVelocityTargetValue=0  RyVelocityTargetValueUnits=deg/s  RyEquilibriumPosition=0  RyEquilibriumPositionUnits=deg  RySpringStiffness=0  RySpringStiffnessUnits=N*m/deg  RyDampingCoefficient=0  RyDampingCoefficientUnits=N*m/(deg/s)  RyLowerLimitSpecify=off  RyLowerLimitBound=-90  RyLowerLimitBoundUnits=deg  RyLowerLimitStiffness=1e4  RyLowerLimitStiffnessUnits=N*m/deg  RyLowerLimitDamping=10  RyLowerLimitDampingUnits=N*m/(deg/s)  RyLowerLimitTransitionRegionWidth=0.1  RyLowerLimitTransitionRegionWidthUnits=deg  RyUpperLimitSpecify=off  RyUpperLimitBound=90  RyUpperLimitBoundUnits=deg  RyUpperLimitStiffness=1e4  RyUpperLimitStiffnessUnits=N*m/deg  RyUpperLimitDamping=10  RyUpperLimitDampingUnits=N*m/(deg/s)  RyUpperLimitTransitionRegionWidth=0.1  RyUpperLimitTransitionRegionWidthUnits=deg  RyTorqueActuationMode=NoTorque  RyMotionActuationMode=ComputedMotion  RySensePosition=off  RySenseVelocity=off  RySenseAcceleration=off  RySenseTorqueForce=off  RySenseLowerLimitTorqueForce=off  RySenseUpperLimitTorqueForce=off
  Universal ToothbarL ActF : sm_lib/Joints/Universal Joint  JointMode=Normal  CompositeWrenchDir=FollowerOnBase  CompositeWrenchFrame=BaseFrame  SenseConstraintForce=off  SenseConstraintTorque=off  SenseTotalForce=off  SenseTotalTorque=off  RxPositionTargetSpecify=off  RxPositionTargetPriority=High  RxPositionTargetValue=0  RxPositionTargetValueUnits=deg  RxVelocityTargetSpecify=off  RxVelocityTargetPriority=High  RxVelocityTargetValue=0  RxVelocityTargetValueUnits=deg/s  RxEquilibriumPosition=0  RxEquilibriumPositionUnits=deg  RxSpringStiffness=0  RxSpringStiffnessUnits=N*m/deg  RxDampingCoefficient=0  RxDampingCoefficientUnits=N*m/(deg/s)  RxLowerLimitSpecify=off  RxLowerLimitBound=-90  RxLowerLimitBoundUnits=deg  RxLowerLimitStiffness=1e4  RxLowerLimitStiffnessUnits=N*m/deg  RxLowerLimitDamping=10  RxLowerLimitDampingUnits=N*m/(deg/s)  RxLowerLimitTransitionRegionWidth=0.1  RxLowerLimitTransitionRegionWidthUnits=deg  RxUpperLimitSpecify=off  RxUpperLimitBound=90  RxUpperLimitBoundUnits=deg  RxUpperLimitStiffness=1e4  RxUpperLimitStiffnessUnits=N*m/deg  RxUpperLimitDamping=10  RxUpperLimitDampingUnits=N*m/(deg/s)  RxUpperLimitTransitionRegionWidth=0.1  RxUpperLimitTransitionRegionWidthUnits=deg  RxTorqueActuationMode=NoTorque  RxMotionActuationMode=ComputedMotion  RxSensePosition=off  RxSenseVelocity=off  RxSenseAcceleration=off  RxSenseTorqueForce=off  RxSenseLowerLimitTorqueForce=off  RxSenseUpperLimitTorqueForce=off  RyPositionTargetSpecify=off  RyPositionTargetPriority=High  RyPositionTargetValue=0  RyPositionTargetValueUnits=deg  RyVelocityTargetSpecify=off  RyVelocityTargetPriority=High  RyVelocityTargetValue=0  RyVelocityTargetValueUnits=deg/s  RyEquilibriumPosition=0  RyEquilibriumPositionUnits=deg  RySpringStiffness=0  RySpringStiffnessUnits=N*m/deg  RyDampingCoefficient=0  RyDampingCoefficientUnits=N*m/(deg/s)  RyLowerLimitSpecify=off  RyLowerLimitBound=-90  RyLowerLimitBoundUnits=deg  RyLowerLimitStiffness=1e4  RyLowerLimitStiffnessUnits=N*m/deg  RyLowerLimitDamping=10  RyLowerLimitDampingUnits=N*m/(deg/s)  RyLowerLimitTransitionRegionWidth=0.1  RyLowerLimitTransitionRegionWidthUnits=deg  RyUpperLimitSpecify=off  RyUpperLimitBound=90  RyUpperLimitBoundUnits=deg  RyUpperLimitStiffness=1e4  RyUpperLimitStiffnessUnits=N*m/deg  RyUpperLimitDamping=10  RyUpperLimitDampingUnits=N*m/(deg/s)  RyUpperLimitTransitionRegionWidth=0.1  RyUpperLimitTransitionRegionWidthUnits=deg  RyTorqueActuationMode=NoTorque  RyMotionActuationMode=ComputedMotion  RySensePosition=off  RySenseVelocity=off  RySenseAcceleration=off  RySenseTorqueForce=off  RySenseLowerLimitTorqueForce=off  RySenseUpperLimitTorqueForce=off
  Universal ToothbarR ActB : sm_lib/Joints/Universal Joint  JointMode=Normal  CompositeWrenchDir=FollowerOnBase  CompositeWrenchFrame=BaseFrame  SenseConstraintForce=off  SenseConstraintTorque=off  SenseTotalForce=off  SenseTotalTorque=off  RxPositionTargetSpecify=off  RxPositionTargetPriority=High  RxPositionTargetValue=0  RxPositionTargetValueUnits=deg  RxVelocityTargetSpecify=off  RxVelocityTargetPriority=High  RxVelocityTargetValue=0  RxVelocityTargetValueUnits=deg/s  RxEquilibriumPosition=0  RxEquilibriumPositionUnits=deg  RxSpringStiffness=0  RxSpringStiffnessUnits=N*m/deg  RxDampingCoefficient=0  RxDampingCoefficientUnits=N*m/(deg/s)  RxLowerLimitSpecify=off  RxLowerLimitBound=-90  RxLowerLimitBoundUnits=deg  RxLowerLimitStiffness=1e4  RxLowerLimitStiffnessUnits=N*m/deg  RxLowerLimitDamping=10  RxLowerLimitDampingUnits=N*m/(deg/s)  RxLowerLimitTransitionRegionWidth=0.1  RxLowerLimitTransitionRegionWidthUnits=deg  RxUpperLimitSpecify=off  RxUpperLimitBound=90  RxUpperLimitBoundUnits=deg  RxUpperLimitStiffness=1e4  RxUpperLimitStiffnessUnits=N*m/deg  RxUpperLimitDamping=10  RxUpperLimitDampingUnits=N*m/(deg/s)  RxUpperLimitTransitionRegionWidth=0.1  RxUpperLimitTransitionRegionWidthUnits=deg  RxTorqueActuationMode=NoTorque  RxMotionActuationMode=ComputedMotion  RxSensePosition=off  RxSenseVelocity=off  RxSenseAcceleration=off  RxSenseTorqueForce=off  RxSenseLowerLimitTorqueForce=off  RxSenseUpperLimitTorqueForce=off  RyPositionTargetSpecify=off  RyPositionTargetPriority=High  RyPositionTargetValue=0  RyPositionTargetValueUnits=deg  RyVelocityTargetSpecify=off  RyVelocityTargetPriority=High  RyVelocityTargetValue=0  RyVelocityTargetValueUnits=deg/s  RyEquilibriumPosition=0  RyEquilibriumPositionUnits=deg  RySpringStiffness=0  RySpringStiffnessUnits=N*m/deg  RyDampingCoefficient=0  RyDampingCoefficientUnits=N*m/(deg/s)  RyLowerLimitSpecify=off  RyLowerLimitBound=-90  RyLowerLimitBoundUnits=deg  RyLowerLimitStiffness=1e4  RyLowerLimitStiffnessUnits=N*m/deg  RyLowerLimitDamping=10  RyLowerLimitDampingUnits=N*m/(deg/s)  RyLowerLimitTransitionRegionWidth=0.1  RyLowerLimitTransitionRegionWidthUnits=deg  RyUpperLimitSpecify=off  RyUpperLimitBound=90  RyUpperLimitBoundUnits=deg  RyUpperLimitStiffness=1e4  RyUpperLimitStiffnessUnits=N*m/deg  RyUpperLimitDamping=10  RyUpperLimitDampingUnits=N*m/(deg/s)  RyUpperLimitTransitionRegionWidth=0.1  RyUpperLimitTransitionRegionWidthUnits=deg  RyTorqueActuationMode=NoTorque  RyMotionActuationMode=ComputedMotion  RySensePosition=off  RySenseVelocity=off  RySenseAcceleration=off  RySenseTorqueForce=off  RySenseLowerLimitTorqueForce=off  RySenseUpperLimitTorqueForce=off
  Universal ToothbarR ActF : sm_lib/Joints/Universal Joint  JointMode=Normal  CompositeWrenchDir=FollowerOnBase  CompositeWrenchFrame=BaseFrame  SenseConstraintForce=off  SenseConstraintTorque=off  SenseTotalForce=off  SenseTotalTorque=off  RxPositionTargetSpecify=off  RxPositionTargetPriority=High  RxPositionTargetValue=0  RxPositionTargetValueUnits=deg  RxVelocityTargetSpecify=off  RxVelocityTargetPriority=High  RxVelocityTargetValue=0  RxVelocityTargetValueUnits=deg/s  RxEquilibriumPosition=0  RxEquilibriumPositionUnits=deg  RxSpringStiffness=0  RxSpringStiffnessUnits=N*m/deg  RxDampingCoefficient=0  RxDampingCoefficientUnits=N*m/(deg/s)  RxLowerLimitSpecify=off  RxLowerLimitBound=-90  RxLowerLimitBoundUnits=deg  RxLowerLimitStiffness=1e4  RxLowerLimitStiffnessUnits=N*m/deg  RxLowerLimitDamping=10  RxLowerLimitDampingUnits=N*m/(deg/s)  RxLowerLimitTransitionRegionWidth=0.1  RxLowerLimitTransitionRegionWidthUnits=deg  RxUpperLimitSpecify=off  RxUpperLimitBound=90  RxUpperLimitBoundUnits=deg  RxUpperLimitStiffness=1e4  RxUpperLimitStiffnessUnits=N*m/deg  RxUpperLimitDamping=10  RxUpperLimitDampingUnits=N*m/(deg/s)  RxUpperLimitTransitionRegionWidth=0.1  RxUpperLimitTransitionRegionWidthUnits=deg  RxTorqueActuationMode=NoTorque  RxMotionActuationMode=ComputedMotion  RxSensePosition=off  RxSenseVelocity=off  RxSenseAcceleration=off  RxSenseTorqueForce=off  RxSenseLowerLimitTorqueForce=off  RxSenseUpperLimitTorqueForce=off  RyPositionTargetSpecify=off  RyPositionTargetPriority=High  RyPositionTargetValue=0  RyPositionTargetValueUnits=deg  RyVelocityTargetSpecify=off  RyVelocityTargetPriority=High  RyVelocityTargetValue=0  RyVelocityTargetValueUnits=deg/s  RyEquilibriumPosition=0  RyEquilibriumPositionUnits=deg  RySpringStiffness=0  RySpringStiffnessUnits=N*m/deg  RyDampingCoefficient=0  RyDampingCoefficientUnits=N*m/(deg/s)  RyLowerLimitSpecify=off  RyLowerLimitBound=-90  RyLowerLimitBoundUnits=deg  RyLowerLimitStiffness=1e4  RyLowerLimitStiffnessUnits=N*m/deg  RyLowerLimitDamping=10  RyLowerLimitDampingUnits=N*m/(deg/s)  RyLowerLimitTransitionRegionWidth=0.1  RyLowerLimitTransitionRegionWidthUnits=deg  RyUpperLimitSpecify=off  RyUpperLimitBound=90  RyUpperLimitBoundUnits=deg  RyUpperLimitStiffness=1e4  RyUpperLimitStiffnessUnits=N*m/deg  RyUpperLimitDamping=10  RyUpperLimitDampingUnits=N*m/(deg/s)  RyUpperLimitTransitionRegionWidth=0.1  RyUpperLimitTransitionRegionWidthUnits=deg  RyTorqueActuationMode=NoTorque  RyMotionActuationMode=ComputedMotion  RySensePosition=off  RySenseVelocity=off  RySenseAcceleration=off  RySenseTorqueForce=off  RySenseLowerLimitTorqueForce=off  RySenseUpperLimitTorqueForce=off
  Act : PMIOPort  Side=Right
  GImpl : PMIOPort  Port=2  Side=Right
  Link : PMIOPort  Port=3  Side=Left
  Arm : PMIOPort  Port=4  Side=Left
  m : Outport
  wires:
  [pR] -> Sum/2
  [pL] -> Sum/1
  Toothbar ActL/2(pwr) -> [pL]
  Bus Creator/1 -> m/1
  [R] -> Bus Selector2/1
  Bus Selector2/3 -> Bus Creator/7  "<pR>"
  Bus Selector2/2 -> Bus Creator/6  "<vR>"
  Bus Selector2/1 -> Bus Creator/5  "<forceR>"
  Bus Selector1/3 -> Bus Creator/3  "<pL>"
  Bus Selector1/2 -> Bus Creator/2  "<vL>"
  Bus Selector1/1 -> Bus Creator/1  "<forceL>"
  [L] -> Bus Selector1/1
  Sum/1 -> Bus Creator/4  "power"
  Toothbar ActR/1(m) -> [R]
  Toothbar ActL/1(m) -> [L]
  Bus Element In1/1 -> Toothbar ActL/1(p)
  Toothbar ActR/2(pwr) -> [pR]
  Bus Element In2/1 -> Toothbar ActR/1(p)
  connections:
  GImpl/RConn1 -- Simscape Bus/RConn1
  Link/RConn1 -- Rake/LConn1
  Point Cloud Toothbar R/RConn1 -- Simscape Bus/LConn3
  Point Cloud Rake/RConn1 -- Simscape Bus/LConn2
  Point Cloud Toothbar L/RConn1 -- Simscape Bus/LConn1
  Rake/RConn1 -- Universal ToothbarL ActB/LConn1
  Toothbar ActL/RConn1 -- Universal ToothbarL ActF/LConn1
  Universal ToothbarL ActF/RConn1 -- LeftToothbar/LConn1
  Rake/RConn5 -- Revolute Toothbar R/LConn1
  Universal ToothbarR ActF/RConn1 -- RightToothbar/LConn1
  Toothbar ActL/LConn2 -- Universal ToothbarL ActB/RConn1
  Revolute Toothbar R/RConn1 -- RightToothbar/LConn2
  Point Cloud Toothbar R/LConn1 -- RightToothbar/RConn1
  Point Cloud Rake/LConn1 -- Rake/RConn3
  Toothbar ActR/RConn1 -- Universal ToothbarR ActF/LConn1
  Rake/RConn2 -- Revolute Toothbar L/LConn1
  Revolute Toothbar L/RConn1 -- LeftToothbar/LConn2
  Arm/RConn1 -- Rake/LConn2
  Rake/RConn4 -- Universal ToothbarR ActB/LConn1
  Point Cloud Toothbar L/LConn1 -- LeftToothbar/RConn1
  Toothbar ActR/LConn2 -- Universal ToothbarR ActB/RConn1
  Connection Label/LConn1 -- Toothbar ActL/LConn1
  Connection Label1/LConn1 -- Toothbar ActR/LConn1
  Simscape Bus1/LConn1 -- Connection Label2/LConn1
  Simscape Bus1/LConn2 -- Connection Label3/LConn1
  Act/RConn1 -- Simscape Bus1/RConn1

== system sm_wheel_loader_lib/Wheel Loader Vehicle/Linkage/Lift Actuator L/Actuator ==
  p : Inport
  Position : Subsystem  VariantControl=Position
      mask Display: image('sm_wheel_loader_cyljoint_Position_IMAGE.png')
  Shaft : Subsystem  VariantControl=Shaft
      mask Display: image('sm_wheel_loader_cyljoint_Shaft_IMAGE.png')
  R : PMIOPort  Side=Left
  B : PMIOPort  Port=2  Side=Left
  F : PMIOPort  Port=3  Side=Right
  m : Outport
